simulink library "quadcopter_propulsion_lib"  (R2018b)
settings: Solver=VariableStepAuto  StartTime=0.0  StopTime=10.0  RelTol=1e-3
undefined symbols (not defined in the file): copterConfig, prop_map_fit, propInertia
libraries: propulsion_lib x4
settings Model: Creator=Ybeyer  LastModifiedBy=yannic
settings SFSimCC: SimUseLocalCustomCode=off
settings RTWCC: RTWUseLocalCustomCode=off
settings CodeAppCC: StateflowObjectComments=on

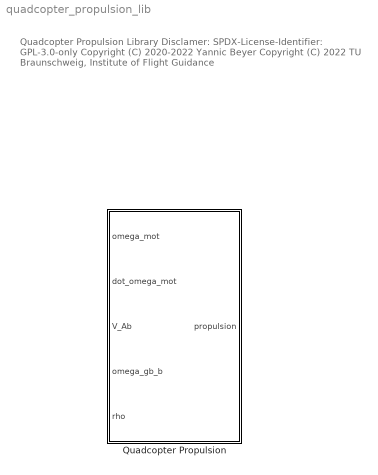
== system quadcopter_propulsion_lib ==
  note: Quadcopter Propulsion Library
      |
      | Disclamer:
      | SPDX-License-Identifier: GPL-3.0-only
      |
      | Copyright (C) 2020-2022 Yannic Beyer
      | Copyright (C) 2022 TU Braunschweig, Institute of Flight Guidance
  Quadcopter Propulsion : Subsystem  mask{copterConfig=copterConfig, map_fit=prop_map_fit, propInertia=propInertia}
      mask prompts: copterConfig "copter configuration struct"; map_fit "propeller map fit (struct), see propMapFitCreate"; propInertia "propeller inertia"
      mask DialogControl DescGroupVar Prompt: Quadcopter Propulsion
      mask DialogControl DescTextVar Prompt: Map-based quadrocopter propulsion.
      mask DialogControl Control2 Prompt: Thrust and torque depend on a map depending on RPM and airspeed perpendicular to the propeller disk.

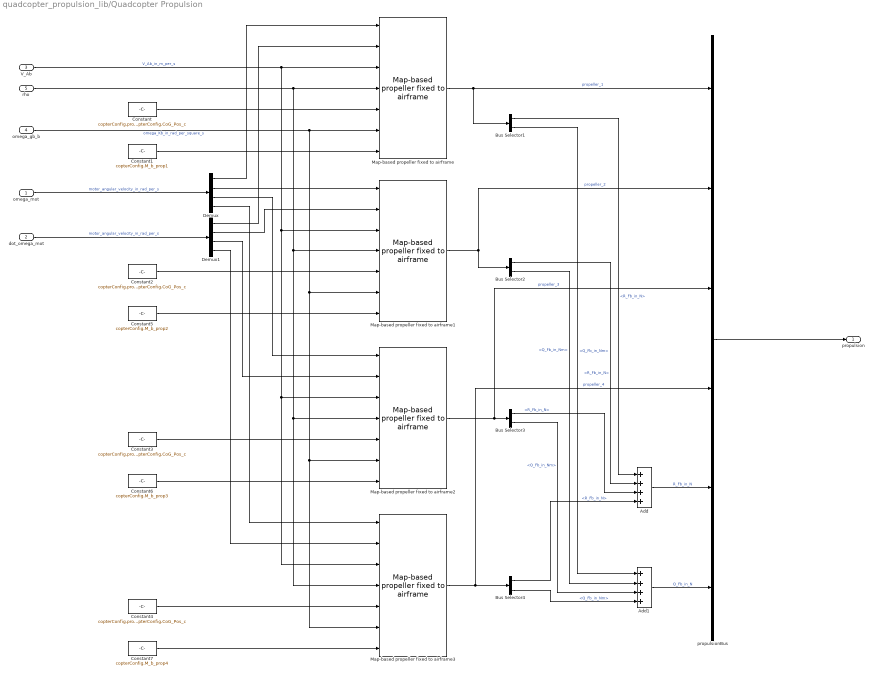
== system quadcopter_propulsion_lib/Quadcopter Propulsion ==
  omega_mot : Inport  PortDimensions=4
  dot_omega_mot : Inport  Port=2  PortDimensions=4
  V_Ab : Inport  Port=3  PortDimensions=3
  "omega_gb_b " : Inport  Port=4  PortDimensions=3
  rho : Inport  Port=5  PortDimensions=1
  Add : Sum  Inputs=4
  Add1 : Sum  Inputs=4
  Bus Selector{1..4} (4 alike) : BusSelector  OutputSignals=R_Fb_in_N,Q_Fb_in_Nm
  Constant : Constant  Value=copterConfig.propPos_c(:,1) - copterConfig.CoG_Pos_c
  Constant1 : Constant  Value=copterConfig.M_b_prop1
  Constant2 : Constant  Value=copterConfig.propPos_c(:,2) - copterConfig.CoG_Pos_c
  Constant3 : Constant  Value=copterConfig.propPos_c(:,3) - copterConfig.CoG_Pos_c
  Constant4 : Constant  Value=copterConfig.propPos_c(:,4) - copterConfig.CoG_Pos_c
  Constant5 : Constant  Value=copterConfig.M_b_prop2
  Constant6 : Constant  Value=copterConfig.M_b_prop3
  Constant7 : Constant  Value=copterConfig.M_b_prop4
  Demux : Demux
  Demux1 : Demux
  Map-based propeller fixed to airframe : propulsion_lib/Map-based propeller fixed to airframe  prop_map_fit=map_fit  I_prop=propInertia  rotation_orientation=copterConfig.propDir(1)
      settings: SourceProductName=LADAC
  Map-based propeller fixed to airframe1 : propulsion_lib/Map-based propeller fixed to airframe  prop_map_fit=map_fit  I_prop=propInertia  rotation_orientation=copterConfig.propDir(2)
      settings: SourceProductName=LADAC
  Map-based propeller fixed to airframe2 : propulsion_lib/Map-based propeller fixed to airframe  prop_map_fit=map_fit  I_prop=propInertia  rotation_orientation=copterConfig.propDir(3)
      settings: SourceProductName=LADAC
  Map-based propeller fixed to airframe3 : propulsion_lib/Map-based propeller fixed to airframe  prop_map_fit=map_fit  I_prop=propInertia  rotation_orientation=copterConfig.propDir(4)
      settings: SourceProductName=LADAC
  propulsionBus : BusCreator  Inputs=6
  propulsion : Outport
  wires:
  Demux1/1 -> Map-based propeller fixed to airframe/2
  V_Ab/1 -> Map-based propeller fixed to airframe3/3, Map-based propeller fixed to airframe2/3, Map-based propeller fixed to airframe1/3, Map-based propeller fixed to airframe/3  "V_Ab_in_m_per_s"
  Constant5/1 -> Map-based propeller fixed to airframe1/7
  Bus Selector1/1 -> Add/1  "<R_Fb_in_N>"
  Constant/1 -> Map-based propeller fixed to airframe/5
  Bus Selector2/1 -> Add/2  "<R_Fb_in_N>"
  Bus Selector1/2 -> Add1/1  "<Q_Fb_in_Nm>"
  Demux1/3 -> Map-based propeller fixed to airframe2/2
  Demux1/4 -> Map-based propeller fixed to airframe3/2
  Bus Selector4/1 -> Add/4  "<R_Fb_in_N>"
  Constant6/1 -> Map-based propeller fixed to airframe2/7
  Bus Selector3/2 -> Add1/3  "<Q_Fb_in_Nm>"
  Demux1/2 -> Map-based propeller fixed to airframe1/2
  Demux/1 -> Map-based propeller fixed to airframe/1
  Constant2/1 -> Map-based propeller fixed to airframe1/5
  Map-based propeller fixed to airframe3/1 -> Bus Selector4/1, propulsionBus/4  "propeller_4"
  propulsionBus/1 -> propulsion/1
  Bus Selector4/2 -> Add1/4  "<Q_Fb_in_Nm>"
  Demux/2 -> Map-based propeller fixed to airframe1/1
  Map-based propeller fixed to airframe1/1 -> Bus Selector2/1, propulsionBus/2  "propeller_2"
  Bus Selector3/1 -> Add/3  "<R_Fb_in_N>"
  Constant7/1 -> Map-based propeller fixed to airframe3/7
  Add/1 -> propulsionBus/5  "R_Fb_in_N"
  "omega_gb_b "/1 -> Map-based propeller fixed to airframe3/6, Map-based propeller fixed to airframe2/6, Map-based propeller fixed to airframe1/6, Map-based propeller fixed to airframe/6  "omega_Kb_in_rad_per_square_s"
  Constant3/1 -> Map-based propeller fixed to airframe2/5
  rho/1 -> Map-based propeller fixed to airframe3/4, Map-based propeller fixed to airframe2/4, Map-based propeller fixed to airframe1/4, Map-based propeller fixed to airframe/4
  Map-based propeller fixed to airframe2/1 -> propulsionBus/3, Bus Selector3/1  "propeller_3"
  Demux/3 -> Map-based propeller fixed to airframe2/1
  Constant1/1 -> Map-based propeller fixed to airframe/7
  Bus Selector2/2 -> Add1/2  "<Q_Fb_in_Nm>"
  Map-based propeller fixed to airframe/1 -> propulsionBus/1, Bus Selector1/1  "propeller_1"
  Add1/1 -> propulsionBus/6  "Q_Fb_in_N"
  Constant4/1 -> Map-based propeller fixed to airframe3/5
  Demux/4 -> Map-based propeller fixed to airframe3/1
  omega_mot/1 -> Demux/1  "motor_angular_velocity_in_rad_per_s"
  dot_omega_mot/1 -> Demux1/1  "motor_angular_velocity_in_rad_per_s"
